simulink model "snap_sys_clk_feng"  (R2019a)
settings: Solver=VariableStepDiscrete  StartTime=0.0  StopTime=10.0  RelTol=1e-3
undefined symbols (not defined in the file): datetime, posixtime
libraries: xbsIndex_r4 x5252, casper_library_misc x69, xps_library x6, casper_library_delays x3
(part 39 of 45)

== system snap_sys_clk_feng/eq/pol1/conv_4bit/round4 ==
  din : Inport
  scale : Inport  Port=2
  Concat1 : xbsIndex_r4/Concat  num_inputs=2  dbl_ovrd=off  block_type=concat
      settings: block_version=10.1.3
  Concat2 : xbsIndex_r4/Concat  num_inputs=2  dbl_ovrd=off  block_type=concat
      settings: block_version=10.1.3
  Constant{,2,4,6} (4 alike) : xbsIndex_r4/Constant  const=(2^n_bits_out - 1) / 2^(n_bits_out)  gui_display_data_type=Fixed-point  arith_type=Signed (2's comp)  n_bits=n_bits_out  bin_pt=n_bits_out-1  preci_type=Single  exp_width=8  frac_width=24  explicit_period=on  period=1  equ=P=C  opselect=C  inp2=PCIN>>17  opr=+  inp1=P  carry=CIN  dbl_ovrd=off  block_type=constant
  Constant{1,3,5,7} (4 alike) : xbsIndex_r4/Constant  const=-(2^n_bits_out - 2) / 2^(n_bits_out)  gui_display_data_type=Fixed-point  arith_type=Signed (2's comp)  n_bits=n_bits_out  bin_pt=n_bits_out-1  preci_type=Single  exp_width=8  frac_width=24  explicit_period=on  period=1  equ=P=C  opselect=C  inp2=PCIN>>17  opr=+  inp1=P  carry=CIN  dbl_ovrd=off  block_type=constant
  Convert : xbsIndex_r4/Convert  gui_display_data_type=Fixed-point  arith_type="Signed  (2's comp)"  n_bits=n_bits_out  bin_pt=n_bits_out-1  float_type=Single  exp_bits=8  fraction_bits=24  quantization="Round  (unbiased: Even Values)"  overflow=Saturate  en=off  latency=5  pipeline=on  dbl_ovrd=off  block_type=convert
  Convert1 : xbsIndex_r4/Convert  gui_display_data_type=Fixed-point  arith_type="Signed  (2's comp)"  n_bits=n_bits_out  bin_pt=n_bits_out-1  float_type=Single  exp_bits=8  fraction_bits=24  quantization="Round  (unbiased: Even Values)"  overflow=Saturate  en=off  latency=5  pipeline=on  dbl_ovrd=off  block_type=convert
  Logical1 : xbsIndex_r4/Logical  logical_function=OR  inputs=4  en=off  latency=1  precision=Full  arith_type=Unsigned  n_bits=8  bin_pt=2  align_bp=on  dbl_ovrd=off  block_type=logical
      settings: xl_area=[0, 0, 0, 0, 0, 0, 0]
  Mult : xbsIndex_r4/Mult  precision=Full  arith_type="Signed  (2's comp)"  n_bits=8  bin_pt=2  quantization=Truncate  overflow=Wrap  en=off  latency=6  use_behavioral_HDL=off  opt=Speed  use_embedded=on  optimum_pipeline=off  pipeline=on  dbl_ovrd=off  use_rpm=on  placement_style=Rectangular shape  block_type=mult
      settings: xl_area=[0, 0, 0, 0, 0, 0, 0]  block_version=10.1.3
  Mult1 : xbsIndex_r4/Mult  precision=Full  arith_type="Signed  (2's comp)"  n_bits=8  bin_pt=2  quantization=Truncate  overflow=Wrap  en=off  latency=6  use_behavioral_HDL=off  opt=Speed  use_embedded=on  optimum_pipeline=on  pipeline=on  dbl_ovrd=off  use_rpm=on  placement_style=Rectangular shape  block_type=mult
      settings: xl_area=[0, 0, 0, 0, 0, 0, 0]  block_version=10.1.3
  Mux : xbsIndex_r4/Mux  inputs=3  en=off  latency=1  precision=Full  arith_type="Signed  (2's comp)"  n_bits=8  bin_pt=2  quantization=Truncate  overflow=Wrap  dbl_ovrd=off  block_type=mux
      settings: xl_area=[0, 0, 0, 0, 0, 0, 0]
  Mux1 : xbsIndex_r4/Mux  inputs=3  en=off  latency=1  precision=Full  arith_type="Signed  (2's comp)"  n_bits=8  bin_pt=2  quantization=Truncate  overflow=Wrap  dbl_ovrd=off  block_type=mux
      settings: xl_area=[0, 0, 0, 0, 0, 0, 0]
  Reinterpret4 : xbsIndex_r4/Reinterpret  force_arith_type=off  arith_type="Signed  (2's comp)"  force_bin_pt=on  bin_pt=coeff_bp  block_type=reinterpret
      settings: block_version=10.1.3
  Relational : xbsIndex_r4/Relational  mode=a>b  op_type=Bool  en=off  latency=5  dbl_ovrd=off  block_type=relational
      settings: xl_area=[0, 0, 0, 0, 0, 0, 0]  block_version=10.1.3
  Relational1 : xbsIndex_r4/Relational  mode=a<b  op_type=Bool  en=off  latency=5  dbl_ovrd=off  block_type=relational
      settings: xl_area=[0, 0, 0, 0, 0, 0, 0]  block_version=10.1.3
  Relational2 : xbsIndex_r4/Relational  mode=a>b  op_type=Bool  en=off  latency=5  dbl_ovrd=off  block_type=relational
      settings: xl_area=[0, 0, 0, 0, 0, 0, 0]  block_version=10.1.3
  Relational3 : xbsIndex_r4/Relational  mode=a<b  op_type=Bool  en=off  latency=5  dbl_ovrd=off  block_type=relational
      settings: xl_area=[0, 0, 0, 0, 0, 0, 0]  block_version=10.1.3
  c_to_ri : casper_library_misc/c_to_ri  n_bits=n_bits_in  bin_pt=n_bits_in-1
      settings: AttributesFormatString=25_24 r/i  SourceProductName=CASPER DSP Blockset
  ri_to_c : casper_library_misc/ri_to_c
      settings: SourceProductName=CASPER DSP Blockset
  dout : Outport
  clip : Outport  Port=2
  wires:
  din/1 -> c_to_ri/1
  ri_to_c/1 -> dout/1
  c_to_ri/1 -> Mult/1
  scale/1 -> Reinterpret4/1
  Convert/1 -> Mux/2
  Concat1/1 -> Mux/1
  Constant/1 -> Relational/2
  Constant1/1 -> Relational1/2
  Constant2/1 -> Mux/3
  Constant3/1 -> Mux/4
  Relational/1 -> Concat1/2, Logical1/1
  Relational1/1 -> Concat1/1, Logical1/2
  Concat2/1 -> Mux1/1
  Constant6/1 -> Mux1/3
  Constant7/1 -> Mux1/4
  Mux/1 -> ri_to_c/1
  Mux1/1 -> ri_to_c/2
  Mult/1 -> Convert/1, Relational/1, Relational1/1
  Logical1/1 -> clip/1
  Reinterpret4/1 -> Mult1/2, Mult/2
  Mult1/1 -> Relational3/1, Relational2/1, Convert1/1
  Constant5/1 -> Relational3/2
  Constant4/1 -> Relational2/2
  Convert1/1 -> Mux1/2
  Relational2/1 -> Logical1/3, Concat2/2
  Relational3/1 -> Logical1/4, Concat2/1
  c_to_ri/2 -> Mult1/1

== system snap_sys_clk_feng/eq/pol1/conv_8bit/bus_expand4 ==
  bus_in : Inport
  reinterpret{1..4} (4 alike) : xbsIndex_r4/Reinterpret  force_arith_type=on  arith_type=Unsigned  force_bin_pt=on  bin_pt=0  block_type=reinterpret
  slice1 : xbsIndex_r4/Slice  nbits=50  boolean_output=off  mode=Upper Bit Location + Width  bit1=-150  base1=MSB of Input  bit0=0  base0=LSB of Input  dbl_ovrd=off  block_type=slice
  slice2 : xbsIndex_r4/Slice  nbits=50  boolean_output=off  mode=Upper Bit Location + Width  bit1=-100  base1=MSB of Input  bit0=0  base0=LSB of Input  dbl_ovrd=off  block_type=slice
  slice3 : xbsIndex_r4/Slice  nbits=50  boolean_output=off  mode=Upper Bit Location + Width  bit1=-50  base1=MSB of Input  bit0=0  base0=LSB of Input  dbl_ovrd=off  block_type=slice
  slice4 : xbsIndex_r4/Slice  nbits=50  boolean_output=off  mode=Upper Bit Location + Width  bit1=0  base1=MSB of Input  bit0=0  base0=LSB of Input  dbl_ovrd=off  block_type=slice
  msb_out4 : Outport
  out3 : Outport  Port=2
  out2 : Outport  Port=3
  lsb_out1 : Outport  Port=4
  wires:
  bus_in/1 -> slice4/1, slice3/1, slice2/1, slice1/1
  slice4/1 -> reinterpret4/1
  reinterpret4/1 -> msb_out4/1
  slice3/1 -> reinterpret3/1
  reinterpret3/1 -> out3/1
  slice2/1 -> reinterpret2/1
  reinterpret2/1 -> out2/1
  slice1/1 -> reinterpret1/1
  reinterpret1/1 -> lsb_out1/1

== system snap_sys_clk_feng/eq/pol1/conv_8bit/round1 ==
  din : Inport
  scale : Inport  Port=2
  Concat1 : xbsIndex_r4/Concat  num_inputs=2  dbl_ovrd=off  block_type=concat
      settings: block_version=10.1.3
  Concat2 : xbsIndex_r4/Concat  num_inputs=2  dbl_ovrd=off  block_type=concat
      settings: block_version=10.1.3
  Constant{,2,4,6} (4 alike) : xbsIndex_r4/Constant  const=(2^n_bits_out - 1) / 2^(n_bits_out)  gui_display_data_type=Fixed-point  arith_type=Signed (2's comp)  n_bits=n_bits_out  bin_pt=n_bits_out-1  preci_type=Single  exp_width=8  frac_width=24  explicit_period=on  period=1  equ=P=C  opselect=C  inp2=PCIN>>17  opr=+  inp1=P  carry=CIN  dbl_ovrd=off  block_type=constant
  Constant{1,3,5,7} (4 alike) : xbsIndex_r4/Constant  const=-(2^n_bits_out - 2) / 2^(n_bits_out)  gui_display_data_type=Fixed-point  arith_type=Signed (2's comp)  n_bits=n_bits_out  bin_pt=n_bits_out-1  preci_type=Single  exp_width=8  frac_width=24  explicit_period=on  period=1  equ=P=C  opselect=C  inp2=PCIN>>17  opr=+  inp1=P  carry=CIN  dbl_ovrd=off  block_type=constant
  Convert : xbsIndex_r4/Convert  gui_display_data_type=Fixed-point  arith_type="Signed  (2's comp)"  n_bits=n_bits_out  bin_pt=n_bits_out-1  float_type=Single  exp_bits=8  fraction_bits=24  quantization="Round  (unbiased: Even Values)"  overflow=Saturate  en=off  latency=5  pipeline=on  dbl_ovrd=off  block_type=convert
  Convert1 : xbsIndex_r4/Convert  gui_display_data_type=Fixed-point  arith_type="Signed  (2's comp)"  n_bits=n_bits_out  bin_pt=n_bits_out-1  float_type=Single  exp_bits=8  fraction_bits=24  quantization="Round  (unbiased: Even Values)"  overflow=Saturate  en=off  latency=5  pipeline=on  dbl_ovrd=off  block_type=convert
  Logical1 : xbsIndex_r4/Logical  logical_function=OR  inputs=4  en=off  latency=1  precision=Full  arith_type=Unsigned  n_bits=8  bin_pt=2  align_bp=on  dbl_ovrd=off  block_type=logical
      settings: xl_area=[0, 0, 0, 0, 0, 0, 0]
  Mult : xbsIndex_r4/Mult  precision=Full  arith_type="Signed  (2's comp)"  n_bits=8  bin_pt=2  quantization=Truncate  overflow=Wrap  en=off  latency=6  use_behavioral_HDL=off  opt=Speed  use_embedded=on  optimum_pipeline=off  pipeline=on  dbl_ovrd=off  use_rpm=on  placement_style=Rectangular shape  block_type=mult
      settings: xl_area=[0, 0, 0, 0, 0, 0, 0]  block_version=10.1.3
  Mult1 : xbsIndex_r4/Mult  precision=Full  arith_type="Signed  (2's comp)"  n_bits=8  bin_pt=2  quantization=Truncate  overflow=Wrap  en=off  latency=6  use_behavioral_HDL=off  opt=Speed  use_embedded=on  optimum_pipeline=on  pipeline=on  dbl_ovrd=off  use_rpm=on  placement_style=Rectangular shape  block_type=mult
      settings: xl_area=[0, 0, 0, 0, 0, 0, 0]  block_version=10.1.3
  Mux : xbsIndex_r4/Mux  inputs=3  en=off  latency=1  precision=Full  arith_type="Signed  (2's comp)"  n_bits=8  bin_pt=2  quantization=Truncate  overflow=Wrap  dbl_ovrd=off  block_type=mux
      settings: xl_area=[0, 0, 0, 0, 0, 0, 0]
  Mux1 : xbsIndex_r4/Mux  inputs=3  en=off  latency=1  precision=Full  arith_type="Signed  (2's comp)"  n_bits=8  bin_pt=2  quantization=Truncate  overflow=Wrap  dbl_ovrd=off  block_type=mux
      settings: xl_area=[0, 0, 0, 0, 0, 0, 0]
  Reinterpret4 : xbsIndex_r4/Reinterpret  force_arith_type=off  arith_type="Signed  (2's comp)"  force_bin_pt=on  bin_pt=coeff_bp  block_type=reinterpret
      settings: block_version=10.1.3
  Relational : xbsIndex_r4/Relational  mode=a>b  op_type=Bool  en=off  latency=5  dbl_ovrd=off  block_type=relational
      settings: xl_area=[0, 0, 0, 0, 0, 0, 0]  block_version=10.1.3
  Relational1 : xbsIndex_r4/Relational  mode=a<b  op_type=Bool  en=off  latency=5  dbl_ovrd=off  block_type=relational
      settings: xl_area=[0, 0, 0, 0, 0, 0, 0]  block_version=10.1.3
  Relational2 : xbsIndex_r4/Relational  mode=a>b  op_type=Bool  en=off  latency=5  dbl_ovrd=off  block_type=relational
      settings: xl_area=[0, 0, 0, 0, 0, 0, 0]  block_version=10.1.3
  Relational3 : xbsIndex_r4/Relational  mode=a<b  op_type=Bool  en=off  latency=5  dbl_ovrd=off  block_type=relational
      settings: xl_area=[0, 0, 0, 0, 0, 0, 0]  block_version=10.1.3
  c_to_ri : casper_library_misc/c_to_ri  n_bits=n_bits_in  bin_pt=n_bits_in-1
      settings: AttributesFormatString=25_24 r/i  SourceProductName=CASPER DSP Blockset
  ri_to_c : casper_library_misc/ri_to_c
      settings: SourceProductName=CASPER DSP Blockset
  dout : Outport
  clip : Outport  Port=2
  wires:
  din/1 -> c_to_ri/1
  ri_to_c/1 -> dout/1
  c_to_ri/1 -> Mult/1
  scale/1 -> Reinterpret4/1
  Convert/1 -> Mux/2
  Concat1/1 -> Mux/1
  Constant/1 -> Relational/2
  Constant1/1 -> Relational1/2
  Constant2/1 -> Mux/3
  Constant3/1 -> Mux/4
  Relational/1 -> Concat1/2, Logical1/1
  Relational1/1 -> Concat1/1, Logical1/2
  Concat2/1 -> Mux1/1
  Constant6/1 -> Mux1/3
  Constant7/1 -> Mux1/4
  Mux/1 -> ri_to_c/1
  Mux1/1 -> ri_to_c/2
  Mult/1 -> Convert/1, Relational/1, Relational1/1
  Logical1/1 -> clip/1
  Reinterpret4/1 -> Mult1/2, Mult/2
  Mult1/1 -> Relational3/1, Relational2/1, Convert1/1
  Constant5/1 -> Relational3/2
  Constant4/1 -> Relational2/2
  Convert1/1 -> Mux1/2
  Relational2/1 -> Logical1/3, Concat2/2
  Relational3/1 -> Logical1/4, Concat2/1
  c_to_ri/2 -> Mult1/1

== system snap_sys_clk_feng/eq/pol1/conv_8bit/round2 ==
  din : Inport
  scale : Inport  Port=2
  Concat1 : xbsIndex_r4/Concat  num_inputs=2  dbl_ovrd=off  block_type=concat
      settings: block_version=10.1.3
  Concat2 : xbsIndex_r4/Concat  num_inputs=2  dbl_ovrd=off  block_type=concat
      settings: block_version=10.1.3
  Constant{,2,4,6} (4 alike) : xbsIndex_r4/Constant  const=(2^n_bits_out - 1) / 2^(n_bits_out)  gui_display_data_type=Fixed-point  arith_type=Signed (2's comp)  n_bits=n_bits_out  bin_pt=n_bits_out-1  preci_type=Single  exp_width=8  frac_width=24  explicit_period=on  period=1  equ=P=C  opselect=C  inp2=PCIN>>17  opr=+  inp1=P  carry=CIN  dbl_ovrd=off  block_type=constant
  Constant{1,3,5,7} (4 alike) : xbsIndex_r4/Constant  const=-(2^n_bits_out - 2) / 2^(n_bits_out)  gui_display_data_type=Fixed-point  arith_type=Signed (2's comp)  n_bits=n_bits_out  bin_pt=n_bits_out-1  preci_type=Single  exp_width=8  frac_width=24  explicit_period=on  period=1  equ=P=C  opselect=C  inp2=PCIN>>17  opr=+  inp1=P  carry=CIN  dbl_ovrd=off  block_type=constant
  Convert : xbsIndex_r4/Convert  gui_display_data_type=Fixed-point  arith_type="Signed  (2's comp)"  n_bits=n_bits_out  bin_pt=n_bits_out-1  float_type=Single  exp_bits=8  fraction_bits=24  quantization="Round  (unbiased: Even Values)"  overflow=Saturate  en=off  latency=5  pipeline=on  dbl_ovrd=off  block_type=convert
  Convert1 : xbsIndex_r4/Convert  gui_display_data_type=Fixed-point  arith_type="Signed  (2's comp)"  n_bits=n_bits_out  bin_pt=n_bits_out-1  float_type=Single  exp_bits=8  fraction_bits=24  quantization="Round  (unbiased: Even Values)"  overflow=Saturate  en=off  latency=5  pipeline=on  dbl_ovrd=off  block_type=convert
  Logical1 : xbsIndex_r4/Logical  logical_function=OR  inputs=4  en=off  latency=1  precision=Full  arith_type=Unsigned  n_bits=8  bin_pt=2  align_bp=on  dbl_ovrd=off  block_type=logical
      settings: xl_area=[0, 0, 0, 0, 0, 0, 0]
  Mult : xbsIndex_r4/Mult  precision=Full  arith_type="Signed  (2's comp)"  n_bits=8  bin_pt=2  quantization=Truncate  overflow=Wrap  en=off  latency=6  use_behavioral_HDL=off  opt=Speed  use_embedded=on  optimum_pipeline=off  pipeline=on  dbl_ovrd=off  use_rpm=on  placement_style=Rectangular shape  block_type=mult
      settings: xl_area=[0, 0, 0, 0, 0, 0, 0]  block_version=10.1.3
  Mult1 : xbsIndex_r4/Mult  precision=Full  arith_type="Signed  (2's comp)"  n_bits=8  bin_pt=2  quantization=Truncate  overflow=Wrap  en=off  latency=6  use_behavioral_HDL=off  opt=Speed  use_embedded=on  optimum_pipeline=on  pipeline=on  dbl_ovrd=off  use_rpm=on  placement_style=Rectangular shape  block_type=mult
      settings: xl_area=[0, 0, 0, 0, 0, 0, 0]  block_version=10.1.3
  Mux : xbsIndex_r4/Mux  inputs=3  en=off  latency=1  precision=Full  arith_type="Signed  (2's comp)"  n_bits=8  bin_pt=2  quantization=Truncate  overflow=Wrap  dbl_ovrd=off  block_type=mux
      settings: xl_area=[0, 0, 0, 0, 0, 0, 0]
  Mux1 : xbsIndex_r4/Mux  inputs=3  en=off  latency=1  precision=Full  arith_type="Signed  (2's comp)"  n_bits=8  bin_pt=2  quantization=Truncate  overflow=Wrap  dbl_ovrd=off  block_type=mux
      settings: xl_area=[0, 0, 0, 0, 0, 0, 0]
  Reinterpret4 : xbsIndex_r4/Reinterpret  force_arith_type=off  arith_type="Signed  (2's comp)"  force_bin_pt=on  bin_pt=coeff_bp  block_type=reinterpret
      settings: block_version=10.1.3
  Relational : xbsIndex_r4/Relational  mode=a>b  op_type=Bool  en=off  latency=5  dbl_ovrd=off  block_type=relational
      settings: xl_area=[0, 0, 0, 0, 0, 0, 0]  block_version=10.1.3
  Relational1 : xbsIndex_r4/Relational  mode=a<b  op_type=Bool  en=off  latency=5  dbl_ovrd=off  block_type=relational
      settings: xl_area=[0, 0, 0, 0, 0, 0, 0]  block_version=10.1.3
  Relational2 : xbsIndex_r4/Relational  mode=a>b  op_type=Bool  en=off  latency=5  dbl_ovrd=off  block_type=relational
      settings: xl_area=[0, 0, 0, 0, 0, 0, 0]  block_version=10.1.3
  Relational3 : xbsIndex_r4/Relational  mode=a<b  op_type=Bool  en=off  latency=5  dbl_ovrd=off  block_type=relational
      settings: xl_area=[0, 0, 0, 0, 0, 0, 0]  block_version=10.1.3
  c_to_ri : casper_library_misc/c_to_ri  n_bits=n_bits_in  bin_pt=n_bits_in-1
      settings: AttributesFormatString=25_24 r/i  SourceProductName=CASPER DSP Blockset
  ri_to_c : casper_library_misc/ri_to_c
      settings: SourceProductName=CASPER DSP Blockset
  dout : Outport
  clip : Outport  Port=2
  wires:
  c_to_ri/2 -> Mult1/1
  Relational3/1 -> Concat2/1, Logical1/4
  Relational2/1 -> Concat2/2, Logical1/3
  Convert1/1 -> Mux1/2
  Constant4/1 -> Relational2/2
  Constant5/1 -> Relational3/2
  Mult1/1 -> Convert1/1, Relational2/1, Relational3/1
  Reinterpret4/1 -> Mult/2, Mult1/2
  Logical1/1 -> clip/1
  Mult/1 -> Relational1/1, Relational/1, Convert/1
  Mux1/1 -> ri_to_c/2
  Mux/1 -> ri_to_c/1
  Constant7/1 -> Mux1/4
  Constant6/1 -> Mux1/3
  Concat2/1 -> Mux1/1
  Relational1/1 -> Logical1/2, Concat1/1
  Relational/1 -> Logical1/1, Concat1/2
  Constant3/1 -> Mux/4
  Constant2/1 -> Mux/3
  Constant1/1 -> Relational1/2
  Constant/1 -> Relational/2
  Concat1/1 -> Mux/1
  Convert/1 -> Mux/2
  scale/1 -> Reinterpret4/1
  c_to_ri/1 -> Mult/1
  ri_to_c/1 -> dout/1
  din/1 -> c_to_ri/1

== system snap_sys_clk_feng/eq/pol1/conv_8bit/round3 ==
  din : Inport
  scale : Inport  Port=2
  Concat1 : xbsIndex_r4/Concat  num_inputs=2  dbl_ovrd=off  block_type=concat
      settings: block_version=10.1.3
  Concat2 : xbsIndex_r4/Concat  num_inputs=2  dbl_ovrd=off  block_type=concat
      settings: block_version=10.1.3
  Constant{,2,4,6} (4 alike) : xbsIndex_r4/Constant  const=(2^n_bits_out - 1) / 2^(n_bits_out)  gui_display_data_type=Fixed-point  arith_type=Signed (2's comp)  n_bits=n_bits_out  bin_pt=n_bits_out-1  preci_type=Single  exp_width=8  frac_width=24  explicit_period=on  period=1  equ=P=C  opselect=C  inp2=PCIN>>17  opr=+  inp1=P  carry=CIN  dbl_ovrd=off  block_type=constant
  Constant{1,3,5,7} (4 alike) : xbsIndex_r4/Constant  const=-(2^n_bits_out - 2) / 2^(n_bits_out)  gui_display_data_type=Fixed-point  arith_type=Signed (2's comp)  n_bits=n_bits_out  bin_pt=n_bits_out-1  preci_type=Single  exp_width=8  frac_width=24  explicit_period=on  period=1  equ=P=C  opselect=C  inp2=PCIN>>17  opr=+  inp1=P  carry=CIN  dbl_ovrd=off  block_type=constant
  Convert : xbsIndex_r4/Convert  gui_display_data_type=Fixed-point  arith_type="Signed  (2's comp)"  n_bits=n_bits_out  bin_pt=n_bits_out-1  float_type=Single  exp_bits=8  fraction_bits=24  quantization="Round  (unbiased: Even Values)"  overflow=Saturate  en=off  latency=5  pipeline=on  dbl_ovrd=off  block_type=convert
  Convert1 : xbsIndex_r4/Convert  gui_display_data_type=Fixed-point  arith_type="Signed  (2's comp)"  n_bits=n_bits_out  bin_pt=n_bits_out-1  float_type=Single  exp_bits=8  fraction_bits=24  quantization="Round  (unbiased: Even Values)"  overflow=Saturate  en=off  latency=5  pipeline=on  dbl_ovrd=off  block_type=convert
  Logical1 : xbsIndex_r4/Logical  logical_function=OR  inputs=4  en=off  latency=1  precision=Full  arith_type=Unsigned  n_bits=8  bin_pt=2  align_bp=on  dbl_ovrd=off  block_type=logical
      settings: xl_area=[0, 0, 0, 0, 0, 0, 0]
  Mult : xbsIndex_r4/Mult  precision=Full  arith_type="Signed  (2's comp)"  n_bits=8  bin_pt=2  quantization=Truncate  overflow=Wrap  en=off  latency=6  use_behavioral_HDL=off  opt=Speed  use_embedded=on  optimum_pipeline=off  pipeline=on  dbl_ovrd=off  use_rpm=on  placement_style=Rectangular shape  block_type=mult
      settings: xl_area=[0, 0, 0, 0, 0, 0, 0]  block_version=10.1.3
  Mult1 : xbsIndex_r4/Mult  precision=Full  arith_type="Signed  (2's comp)"  n_bits=8  bin_pt=2  quantization=Truncate  overflow=Wrap  en=off  latency=6  use_behavioral_HDL=off  opt=Speed  use_embedded=on  optimum_pipeline=on  pipeline=on  dbl_ovrd=off  use_rpm=on  placement_style=Rectangular shape  block_type=mult
      settings: xl_area=[0, 0, 0, 0, 0, 0, 0]  block_version=10.1.3
  Mux : xbsIndex_r4/Mux  inputs=3  en=off  latency=1  precision=Full  arith_type="Signed  (2's comp)"  n_bits=8  bin_pt=2  quantization=Truncate  overflow=Wrap  dbl_ovrd=off  block_type=mux
      settings: xl_area=[0, 0, 0, 0, 0, 0, 0]
  Mux1 : xbsIndex_r4/Mux  inputs=3  en=off  latency=1  precision=Full  arith_type="Signed  (2's comp)"  n_bits=8  bin_pt=2  quantization=Truncate  overflow=Wrap  dbl_ovrd=off  block_type=mux
      settings: xl_area=[0, 0, 0, 0, 0, 0, 0]
  Reinterpret4 : xbsIndex_r4/Reinterpret  force_arith_type=off  arith_type="Signed  (2's comp)"  force_bin_pt=on  bin_pt=coeff_bp  block_type=reinterpret
      settings: block_version=10.1.3
  Relational : xbsIndex_r4/Relational  mode=a>b  op_type=Bool  en=off  latency=5  dbl_ovrd=off  block_type=relational
      settings: xl_area=[0, 0, 0, 0, 0, 0, 0]  block_version=10.1.3
  Relational1 : xbsIndex_r4/Relational  mode=a<b  op_type=Bool  en=off  latency=5  dbl_ovrd=off  block_type=relational
      settings: xl_area=[0, 0, 0, 0, 0, 0, 0]  block_version=10.1.3
  Relational2 : xbsIndex_r4/Relational  mode=a>b  op_type=Bool  en=off  latency=5  dbl_ovrd=off  block_type=relational
      settings: xl_area=[0, 0, 0, 0, 0, 0, 0]  block_version=10.1.3
  Relational3 : xbsIndex_r4/Relational  mode=a<b  op_type=Bool  en=off  latency=5  dbl_ovrd=off  block_type=relational
      settings: xl_area=[0, 0, 0, 0, 0, 0, 0]  block_version=10.1.3
  c_to_ri : casper_library_misc/c_to_ri  n_bits=n_bits_in  bin_pt=n_bits_in-1
      settings: AttributesFormatString=25_24 r/i  SourceProductName=CASPER DSP Blockset
  ri_to_c : casper_library_misc/ri_to_c
      settings: SourceProductName=CASPER DSP Blockset
  dout : Outport
  clip : Outport  Port=2
  wires:
  din/1 -> c_to_ri/1
  ri_to_c/1 -> dout/1
  c_to_ri/1 -> Mult/1
  scale/1 -> Reinterpret4/1
  Convert/1 -> Mux/2
  Concat1/1 -> Mux/1
  Constant/1 -> Relational/2
  Constant1/1 -> Relational1/2
  Constant2/1 -> Mux/3
  Constant3/1 -> Mux/4
  Relational/1 -> Concat1/2, Logical1/1
  Relational1/1 -> Concat1/1, Logical1/2
  Concat2/1 -> Mux1/1
  Constant6/1 -> Mux1/3
  Constant7/1 -> Mux1/4
  Mux/1 -> ri_to_c/1
  Mux1/1 -> ri_to_c/2
  Mult/1 -> Convert/1, Relational/1, Relational1/1
  Logical1/1 -> clip/1
  Reinterpret4/1 -> Mult1/2, Mult/2
  Mult1/1 -> Relational3/1, Relational2/1, Convert1/1
  Constant5/1 -> Relational3/2
  Constant4/1 -> Relational2/2
  Convert1/1 -> Mux1/2
  Relational2/1 -> Logical1/3, Concat2/2
  Relational3/1 -> Logical1/4, Concat2/1
  c_to_ri/2 -> Mult1/1

== system snap_sys_clk_feng/eq/pol1/conv_8bit/round4 ==
  din : Inport
  scale : Inport  Port=2
  Concat1 : xbsIndex_r4/Concat  num_inputs=2  dbl_ovrd=off  block_type=concat
      settings: block_version=10.1.3
  Concat2 : xbsIndex_r4/Concat  num_inputs=2  dbl_ovrd=off  block_type=concat
      settings: block_version=10.1.3
  Constant{,2,4,6} (4 alike) : xbsIndex_r4/Constant  const=(2^n_bits_out - 1) / 2^(n_bits_out)  gui_display_data_type=Fixed-point  arith_type=Signed (2's comp)  n_bits=n_bits_out  bin_pt=n_bits_out-1  preci_type=Single  exp_width=8  frac_width=24  explicit_period=on  period=1  equ=P=C  opselect=C  inp2=PCIN>>17  opr=+  inp1=P  carry=CIN  dbl_ovrd=off  block_type=constant
  Constant{1,3,5,7} (4 alike) : xbsIndex_r4/Constant  const=-(2^n_bits_out - 2) / 2^(n_bits_out)  gui_display_data_type=Fixed-point  arith_type=Signed (2's comp)  n_bits=n_bits_out  bin_pt=n_bits_out-1  preci_type=Single  exp_width=8  frac_width=24  explicit_period=on  period=1  equ=P=C  opselect=C  inp2=PCIN>>17  opr=+  inp1=P  carry=CIN  dbl_ovrd=off  block_type=constant
  Convert : xbsIndex_r4/Convert  gui_display_data_type=Fixed-point  arith_type="Signed  (2's comp)"  n_bits=n_bits_out  bin_pt=n_bits_out-1  float_type=Single  exp_bits=8  fraction_bits=24  quantization="Round  (unbiased: Even Values)"  overflow=Saturate  en=off  latency=5  pipeline=on  dbl_ovrd=off  block_type=convert
  Convert1 : xbsIndex_r4/Convert  gui_display_data_type=Fixed-point  arith_type="Signed  (2's comp)"  n_bits=n_bits_out  bin_pt=n_bits_out-1  float_type=Single  exp_bits=8  fraction_bits=24  quantization="Round  (unbiased: Even Values)"  overflow=Saturate  en=off  latency=5  pipeline=on  dbl_ovrd=off  block_type=convert
  Logical1 : xbsIndex_r4/Logical  logical_function=OR  inputs=4  en=off  latency=1  precision=Full  arith_type=Unsigned  n_bits=8  bin_pt=2  align_bp=on  dbl_ovrd=off  block_type=logical
      settings: xl_area=[0, 0, 0, 0, 0, 0, 0]
  Mult : xbsIndex_r4/Mult  precision=Full  arith_type="Signed  (2's comp)"  n_bits=8  bin_pt=2  quantization=Truncate  overflow=Wrap  en=off  latency=6  use_behavioral_HDL=off  opt=Speed  use_embedded=on  optimum_pipeline=off  pipeline=on  dbl_ovrd=off  use_rpm=on  placement_style=Rectangular shape  block_type=mult
      settings: xl_area=[0, 0, 0, 0, 0, 0, 0]  block_version=10.1.3
  Mult1 : xbsIndex_r4/Mult  precision=Full  arith_type="Signed  (2's comp)"  n_bits=8  bin_pt=2  quantization=Truncate  overflow=Wrap  en=off  latency=6  use_behavioral_HDL=off  opt=Speed  use_embedded=on  optimum_pipeline=on  pipeline=on  dbl_ovrd=off  use_rpm=on  placement_style=Rectangular shape  block_type=mult
      settings: xl_area=[0, 0, 0, 0, 0, 0, 0]  block_version=10.1.3
  Mux : xbsIndex_r4/Mux  inputs=3  en=off  latency=1  precision=Full  arith_type="Signed  (2's comp)"  n_bits=8  bin_pt=2  quantization=Truncate  overflow=Wrap  dbl_ovrd=off  block_type=mux
      settings: xl_area=[0, 0, 0, 0, 0, 0, 0]
  Mux1 : xbsIndex_r4/Mux  inputs=3  en=off  latency=1  precision=Full  arith_type="Signed  (2's comp)"  n_bits=8  bin_pt=2  quantization=Truncate  overflow=Wrap  dbl_ovrd=off  block_type=mux
      settings: xl_area=[0, 0, 0, 0, 0, 0, 0]
  Reinterpret4 : xbsIndex_r4/Reinterpret  force_arith_type=off  arith_type="Signed  (2's comp)"  force_bin_pt=on  bin_pt=coeff_bp  block_type=reinterpret
      settings: block_version=10.1.3
  Relational : xbsIndex_r4/Relational  mode=a>b  op_type=Bool  en=off  latency=5  dbl_ovrd=off  block_type=relational
      settings: xl_area=[0, 0, 0, 0, 0, 0, 0]  block_version=10.1.3
  Relational1 : xbsIndex_r4/Relational  mode=a<b  op_type=Bool  en=off  latency=5  dbl_ovrd=off  block_type=relational
      settings: xl_area=[0, 0, 0, 0, 0, 0, 0]  block_version=10.1.3
  Relational2 : xbsIndex_r4/Relational  mode=a>b  op_type=Bool  en=off  latency=5  dbl_ovrd=off  block_type=relational
      settings: xl_area=[0, 0, 0, 0, 0, 0, 0]  block_version=10.1.3
  Relational3 : xbsIndex_r4/Relational  mode=a<b  op_type=Bool  en=off  latency=5  dbl_ovrd=off  block_type=relational
      settings: xl_area=[0, 0, 0, 0, 0, 0, 0]  block_version=10.1.3
  c_to_ri : casper_library_misc/c_to_ri  n_bits=n_bits_in  bin_pt=n_bits_in-1
      settings: AttributesFormatString=25_24 r/i  SourceProductName=CASPER DSP Blockset
  ri_to_c : casper_library_misc/ri_to_c
      settings: SourceProductName=CASPER DSP Blockset
  dout : Outport
  clip : Outport  Port=2
  wires:
  c_to_ri/2 -> Mult1/1
  Relational3/1 -> Concat2/1, Logical1/4
  Relational2/1 -> Concat2/2, Logical1/3
  Convert1/1 -> Mux1/2
  Constant4/1 -> Relational2/2
  Constant5/1 -> Relational3/2
  Mult1/1 -> Convert1/1, Relational2/1, Relational3/1
  Reinterpret4/1 -> Mult/2, Mult1/2
  Logical1/1 -> clip/1
  Mult/1 -> Relational1/1, Relational/1, Convert/1
  Mux1/1 -> ri_to_c/2
  Mux/1 -> ri_to_c/1
  Constant7/1 -> Mux1/4
  Constant6/1 -> Mux1/3
  Concat2/1 -> Mux1/1
  Relational1/1 -> Logical1/2, Concat1/1
  Relational/1 -> Logical1/1, Concat1/2
  Constant3/1 -> Mux/4
  Constant2/1 -> Mux/3
  Constant1/1 -> Relational1/2
  Constant/1 -> Relational/2
  Concat1/1 -> Mux/1
  Convert/1 -> Mux/2
  scale/1 -> Reinterpret4/1
  c_to_ri/1 -> Mult/1
  ri_to_c/1 -> dout/1
  din/1 -> c_to_ri/1

== system snap_sys_clk_feng/eqtvg/pol0/tv/calc_add ==
  note: If reading/writing words
      | smaller than 32 bits,
      | change address so
      | that addressing is
      | big endian instead of
      | little, otherwise
      | pass through
  note: Use behavioural HDL
      | so that gets optimised
      | to minimum logic
  in : Inport
  add_sub : xbsIndex_r4/AddSub  mode=Subtraction  use_carryin=off  use_carryout=off  en=off  latency=0  precision=User Defined  arith_type=Unsigned  n_bits=max(1, log2(32/data_width))  bin_pt=0  quantization=Truncate  overflow=Wrap  use_behavioral_HDL=on  hw_selection=Fabric  pipelined=off  dbl_ovrd=off  block_type=addsub
  concat : xbsIndex_r4/Concat  num_inputs=2  dbl_ovrd=off  block_type=concat
  const : xbsIndex_r4/Constant  const=max(0, 32/data_width-1)  gui_display_data_type=Fixed-point  arith_type=Unsigned  n_bits=max(1, log2(32/data_width))  bin_pt=0  preci_type=Single  exp_width=8  frac_width=24  explicit_period=on  period=sample_rate  equ=P=C  opselect=C  inp2=PCIN>>17  opr=+  inp1=P  carry=CIN  dbl_ovrd=off  block_type=constant
      settings: block_version=11.4
  convert_addr : xbsIndex_r4/Convert  gui_display_data_type=Fixed-point  arith_type=Unsigned  n_bits=addr_width  bin_pt=0  float_type=Single  exp_bits=8  fraction_bits=24  quantization=Truncate  overflow=Wrap  en=off  latency=0  pipeline=off  dbl_ovrd=off  block_type=convert
      settings: xl_area=[0, 0, 0, 0, 0, 0, 0]
  lsw : xbsIndex_r4/Slice  nbits=max(1, log2(32/data_width))  boolean_output=off  mode=Lower Bit Location + Width  bit1=0  base1=MSB of Input  bit0=0  base0=LSB of Input  dbl_ovrd=off  block_type=slice
  manipulate : xbsIndex_r4/Constant  const=min(1, floor(32/data_width) - 1)  gui_display_data_type=Fixed-point  arith_type=Unsigned  n_bits=1  bin_pt=0  preci_type=Single  exp_width=8  frac_width=24  explicit_period=on  period=sample_rate  equ=P=C  opselect=C  inp2=PCIN>>17  opr=+  inp1=P  carry=CIN  dbl_ovrd=off  block_type=constant
      settings: block_version=11.4
  msw : xbsIndex_r4/Slice  nbits=addr_width - max(1, log2(32/data_width))  boolean_output=off  mode=Upper Bit Location + Width  bit1=0  base1=MSB of Input  bit0=0  base0=LSB of Input  dbl_ovrd=off  block_type=slice
  mux : xbsIndex_r4/Mux  inputs=2  en=off  latency=0  precision=Full  arith_type=Unsigned  n_bits=16  bin_pt=14  quantization=Truncate  overflow=Wrap  dbl_ovrd=off  block_type=mux
      settings: block_version=11.4
  out : Outport
  wires:
  in/1 -> convert_addr/1
  add_sub/1 -> concat/2
  msw/1 -> concat/1
  concat/1 -> mux/3
  manipulate/1 -> mux/1
  mux/1 -> out/1
  lsw/1 -> add_sub/2
  const/1 -> add_sub/1
  convert_addr/1 -> lsw/1, msw/1, mux/2

== system snap_sys_clk_feng/eqtvg/pol0/tv/munge_in ==
  din : Inport
  reinterpret_out : xbsIndex_r4/Reinterpret  force_arith_type=on  arith_type=Unsigned  force_bin_pt=on  bin_pt=0  block_type=reinterpret
  dout : Outport
  wires:
  reinterpret_out/1 -> dout/1
  din/1 -> reinterpret_out/1

== system snap_sys_clk_feng/eqtvg/pol0/tv/munge_out ==
  din : Inport
  reinterpret_out : xbsIndex_r4/Reinterpret  force_arith_type=on  arith_type=Unsigned  force_bin_pt=on  bin_pt=0  block_type=reinterpret
  dout : Outport
  wires:
  reinterpret_out/1 -> dout/1
  din/1 -> reinterpret_out/1

== system snap_sys_clk_feng/eqtvg/pol0/tv/sim_mem ==
  addr : Inport
  data : Inport  Port=2
  we : Inport  Port=3
  Data Type Conversion : DataTypeConversion  OutDataTypeStr=single
  Data Type Conversion1 : DataTypeConversion  OutDataTypeStr=double
  Data Type Conversion2 : DataTypeConversion  OutDataTypeStr=boolean
  sfunc : M-S-Function  FunctionName=shared_bram_sim_sfunc  Parameters=depth_bits, latency, init_vals  mask{depth_bits=addr_width, latency=csp_latency, init_vals=init_vals}
      mask prompts: depth_bits "Depth (2^?):"; latency "Latency (>=1):"; init_vals "Initial values:"
      mask Callback latency:
      | latency = str2double(get_param(gcb, 'latency'));
      | if latency < 1
      |     errordlg('Cannot have latency less than one.');
      |     set_param(gcb, 'latency', '1');
      | end
  sim_addr : xbsIndex_r4/Gateway Out  inherit_from_input=off  hdl_port=off  rows=1  columns=1  UseAsDAC=off  DACChannel='1'  interface=None  automatic_assignment=on  address_offset=hex2dec('00')  intf_name=''  intf_description=''  timing_constraint=None  locs_specified=off  LOCs={}  io_standard={}  block_type=gatewayout
  sim_data : xbsIndex_r4/Gateway Out  inherit_from_input=off  hdl_port=off  rows=1  columns=1  UseAsDAC=off  DACChannel='1'  interface=None  automatic_assignment=on  address_offset=hex2dec('00')  intf_name=''  intf_description=''  timing_constraint=None  locs_specified=off  LOCs={}  io_standard={}  block_type=gatewayout
  sim_we : xbsIndex_r4/Gateway Out  inherit_from_input=off  hdl_port=off  rows=1  columns=1  UseAsDAC=off  DACChannel='1'  interface=None  automatic_assignment=on  address_offset=hex2dec('00')  intf_name=''  intf_description=''  timing_constraint=None  locs_specified=off  LOCs={}  io_standard={}  block_type=gatewayout
  data_out : Outport
  wires:
  addr/1 -> sim_addr/1
  data/1 -> sim_data/1
  we/1 -> sim_we/1
  sim_addr/1 -> Data Type Conversion/1
  sim_data/1 -> Data Type Conversion1/1
  sim_we/1 -> Data Type Conversion2/1
  Data Type Conversion/1 -> sfunc/1  "addr"
  Data Type Conversion1/1 -> sfunc/2  "data_in"
  Data Type Conversion2/1 -> sfunc/3  "we"
  sfunc/1 -> data_out/1  "output"

== system snap_sys_clk_feng/eqtvg/pol1/tv/calc_add ==
  note: Use behavioural HDL
      | so that gets optimised
      | to minimum logic
  note: If reading/writing words
      | smaller than 32 bits,
      | change address so
      | that addressing is
      | big endian instead of
      | little, otherwise
      | pass through
  in : Inport
  add_sub : xbsIndex_r4/AddSub  mode=Subtraction  use_carryin=off  use_carryout=off  en=off  latency=0  precision=User Defined  arith_type=Unsigned  n_bits=max(1, log2(32/data_width))  bin_pt=0  quantization=Truncate  overflow=Wrap  use_behavioral_HDL=on  hw_selection=Fabric  pipelined=off  dbl_ovrd=off  block_type=addsub
  concat : xbsIndex_r4/Concat  num_inputs=2  dbl_ovrd=off  block_type=concat
  const : xbsIndex_r4/Constant  const=max(0, 32/data_width-1)  gui_display_data_type=Fixed-point  arith_type=Unsigned  n_bits=max(1, log2(32/data_width))  bin_pt=0  preci_type=Single  exp_width=8  frac_width=24  explicit_period=on  period=sample_rate  equ=P=C  opselect=C  inp2=PCIN>>17  opr=+  inp1=P  carry=CIN  dbl_ovrd=off  block_type=constant
      settings: block_version=11.4
  convert_addr : xbsIndex_r4/Convert  gui_display_data_type=Fixed-point  arith_type=Unsigned  n_bits=addr_width  bin_pt=0  float_type=Single  exp_bits=8  fraction_bits=24  quantization=Truncate  overflow=Wrap  en=off  latency=0  pipeline=off  dbl_ovrd=off  block_type=convert
      settings: xl_area=[0, 0, 0, 0, 0, 0, 0]
  lsw : xbsIndex_r4/Slice  nbits=max(1, log2(32/data_width))  boolean_output=off  mode=Lower Bit Location + Width  bit1=0  base1=MSB of Input  bit0=0  base0=LSB of Input  dbl_ovrd=off  block_type=slice
  manipulate : xbsIndex_r4/Constant  const=min(1, floor(32/data_width) - 1)  gui_display_data_type=Fixed-point  arith_type=Unsigned  n_bits=1  bin_pt=0  preci_type=Single  exp_width=8  frac_width=24  explicit_period=on  period=sample_rate  equ=P=C  opselect=C  inp2=PCIN>>17  opr=+  inp1=P  carry=CIN  dbl_ovrd=off  block_type=constant
      settings: block_version=11.4
  msw : xbsIndex_r4/Slice  nbits=addr_width - max(1, log2(32/data_width))  boolean_output=off  mode=Upper Bit Location + Width  bit1=0  base1=MSB of Input  bit0=0  base0=LSB of Input  dbl_ovrd=off  block_type=slice
  mux : xbsIndex_r4/Mux  inputs=2  en=off  latency=0  precision=Full  arith_type=Unsigned  n_bits=16  bin_pt=14  quantization=Truncate  overflow=Wrap  dbl_ovrd=off  block_type=mux
      settings: block_version=11.4
  out : Outport
  wires:
  convert_addr/1 -> mux/2, msw/1, lsw/1
  const/1 -> add_sub/1
  lsw/1 -> add_sub/2
  mux/1 -> out/1
  manipulate/1 -> mux/1
  concat/1 -> mux/3
  msw/1 -> concat/1
  add_sub/1 -> concat/2
  in/1 -> convert_addr/1

== system snap_sys_clk_feng/eqtvg/pol1/tv/munge_in ==
  din : Inport
  reinterpret_out : xbsIndex_r4/Reinterpret  force_arith_type=on  arith_type=Unsigned  force_bin_pt=on  bin_pt=0  block_type=reinterpret
  dout : Outport
  wires:
  din/1 -> reinterpret_out/1
  reinterpret_out/1 -> dout/1

== system snap_sys_clk_feng/eqtvg/pol1/tv/munge_out ==
  din : Inport
  reinterpret_out : xbsIndex_r4/Reinterpret  force_arith_type=on  arith_type=Unsigned  force_bin_pt=on  bin_pt=0  block_type=reinterpret
  dout : Outport
  wires:
  din/1 -> reinterpret_out/1
  reinterpret_out/1 -> dout/1

== system snap_sys_clk_feng/eqtvg/pol1/tv/sim_mem ==
  addr : Inport
  data : Inport  Port=2
  we : Inport  Port=3
  Data Type Conversion : DataTypeConversion  OutDataTypeStr=single
  Data Type Conversion1 : DataTypeConversion  OutDataTypeStr=double
  Data Type Conversion2 : DataTypeConversion  OutDataTypeStr=boolean
  sfunc : M-S-Function  FunctionName=shared_bram_sim_sfunc  Parameters=depth_bits, latency, init_vals  mask{depth_bits=addr_width, latency=csp_latency, init_vals=init_vals}
      mask prompts: depth_bits "Depth (2^?):"; latency "Latency (>=1):"; init_vals "Initial values:"
      mask Callback latency:
      | latency = str2double(get_param(gcb, 'latency'));
      | if latency < 1
      |     errordlg('Cannot have latency less than one.');
      |     set_param(gcb, 'latency', '1');
      | end
  sim_addr : xbsIndex_r4/Gateway Out  inherit_from_input=off  hdl_port=off  rows=1  columns=1  UseAsDAC=off  DACChannel='1'  interface=None  automatic_assignment=on  address_offset=hex2dec('00')  intf_name=''  intf_description=''  timing_constraint=None  locs_specified=off  LOCs={}  io_standard={}  block_type=gatewayout
  sim_data : xbsIndex_r4/Gateway Out  inherit_from_input=off  hdl_port=off  rows=1  columns=1  UseAsDAC=off  DACChannel='1'  interface=None  automatic_assignment=on  address_offset=hex2dec('00')  intf_name=''  intf_description=''  timing_constraint=None  locs_specified=off  LOCs={}  io_standard={}  block_type=gatewayout
  sim_we : xbsIndex_r4/Gateway Out  inherit_from_input=off  hdl_port=off  rows=1  columns=1  UseAsDAC=off  DACChannel='1'  interface=None  automatic_assignment=on  address_offset=hex2dec('00')  intf_name=''  intf_description=''  timing_constraint=None  locs_specified=off  LOCs={}  io_standard={}  block_type=gatewayout
  data_out : Outport
  wires:
  sfunc/1 -> data_out/1  "output"
  Data Type Conversion2/1 -> sfunc/3  "we"
  Data Type Conversion1/1 -> sfunc/2  "data_in"
  Data Type Conversion/1 -> sfunc/1  "addr"
  sim_we/1 -> Data Type Conversion2/1
  sim_data/1 -> Data Type Conversion1/1
  sim_addr/1 -> Data Type Conversion/1
  we/1 -> sim_we/1
  data/1 -> sim_data/1
  addr/1 -> sim_addr/1

== system snap_sys_clk_feng/packetizer0/header/munge_in/join ==
  in1 : Inport
  in2 : Inport  Port=2
  concatenate : xbsIndex_r4/Concat  num_inputs=2  dbl_ovrd=off  block_type=concat
  reinterpret1 : xbsIndex_r4/Reinterpret  force_arith_type=on  arith_type=Unsigned  force_bin_pt=on  bin_pt=0  block_type=reinterpret
      settings: infoedit="Changes signal type without altering the binary representation.   You can changed the signal between signed and unsigned, and relocate the binary point.<br><br>Hardware notes: In hardware this block costs nothing.<br><br>Example:  Suppose the input is 6 bits wide, signed, with 2 fractional bits, and the output is forced to unsigned with 0 fractional bits.  Then an input of -2.0 (1110.00 in binary 2's complement) becomes an output of 56 (111000 in binary)."
  reinterpret2 : xbsIndex_r4/Reinterpret  force_arith_type=on  arith_type=Unsigned  force_bin_pt=on  bin_pt=0  block_type=reinterpret
      settings: infoedit="Changes signal type without altering the binary representation.   You can changed the signal between signed and unsigned, and relocate the binary point.<br><br>Hardware notes: In hardware this block costs nothing.<br><br>Example:  Suppose the input is 6 bits wide, signed, with 2 fractional bits, and the output is forced to unsigned with 0 fractional bits.  Then an input of -2.0 (1110.00 in binary 2's complement) becomes an output of 56 (111000 in binary)."
  bus_out : Outport
  wires:
  concatenate/1 -> bus_out/1
  in1/1 -> reinterpret1/1
  reinterpret1/1 -> concatenate/1
  in2/1 -> reinterpret2/1
  reinterpret2/1 -> concatenate/2

== system snap_sys_clk_feng/packetizer0/header/munge_in/split ==
  bus_in : Inport
  reinterpret1 : xbsIndex_r4/Reinterpret  force_arith_type=on  arith_type=Unsigned  force_bin_pt=on  bin_pt=0  block_type=reinterpret
  reinterpret2 : xbsIndex_r4/Reinterpret  force_arith_type=on  arith_type=Unsigned  force_bin_pt=on  bin_pt=0  block_type=reinterpret
  slice1 : xbsIndex_r4/Slice  nbits=32  boolean_output=off  mode=Upper Bit Location + Width  bit1=-32  base1=MSB of Input  bit0=0  base0=LSB of Input  dbl_ovrd=off  block_type=slice
  slice2 : xbsIndex_r4/Slice  nbits=32  boolean_output=off  mode=Upper Bit Location + Width  bit1=0  base1=MSB of Input  bit0=0  base0=LSB of Input  dbl_ovrd=off  block_type=slice
  msb_out2 : Outport
  lsb_out1 : Outport  Port=2
  wires:
  bus_in/1 -> slice2/1, slice1/1
  slice2/1 -> reinterpret2/1
  reinterpret2/1 -> msb_out2/1
  slice1/1 -> reinterpret1/1
  reinterpret1/1 -> lsb_out1/1

== system snap_sys_clk_feng/packetizer0/header/munge_out/join ==
  in1 : Inport
  in2 : Inport  Port=2
  concatenate : xbsIndex_r4/Concat  num_inputs=2  dbl_ovrd=off  block_type=concat
  reinterpret1 : xbsIndex_r4/Reinterpret  force_arith_type=on  arith_type=Unsigned  force_bin_pt=on  bin_pt=0  block_type=reinterpret
      settings: infoedit="Changes signal type without altering the binary representation.   You can changed the signal between signed and unsigned, and relocate the binary point.<br><br>Hardware notes: In hardware this block costs nothing.<br><br>Example:  Suppose the input is 6 bits wide, signed, with 2 fractional bits, and the output is forced to unsigned with 0 fractional bits.  Then an input of -2.0 (1110.00 in binary 2's complement) becomes an output of 56 (111000 in binary)."
  reinterpret2 : xbsIndex_r4/Reinterpret  force_arith_type=on  arith_type=Unsigned  force_bin_pt=on  bin_pt=0  block_type=reinterpret
      settings: infoedit="Changes signal type without altering the binary representation.   You can changed the signal between signed and unsigned, and relocate the binary point.<br><br>Hardware notes: In hardware this block costs nothing.<br><br>Example:  Suppose the input is 6 bits wide, signed, with 2 fractional bits, and the output is forced to unsigned with 0 fractional bits.  Then an input of -2.0 (1110.00 in binary 2's complement) becomes an output of 56 (111000 in binary)."
  bus_out : Outport
  wires:
  concatenate/1 -> bus_out/1
  in1/1 -> reinterpret1/1
  reinterpret1/1 -> concatenate/1
  in2/1 -> reinterpret2/1
  reinterpret2/1 -> concatenate/2

== system snap_sys_clk_feng/packetizer0/header/munge_out/split ==
  bus_in : Inport
  reinterpret1 : xbsIndex_r4/Reinterpret  force_arith_type=on  arith_type=Unsigned  force_bin_pt=on  bin_pt=0  block_type=reinterpret
  reinterpret2 : xbsIndex_r4/Reinterpret  force_arith_type=on  arith_type=Unsigned  force_bin_pt=on  bin_pt=0  block_type=reinterpret
  slice1 : xbsIndex_r4/Slice  nbits=32  boolean_output=off  mode=Upper Bit Location + Width  bit1=-32  base1=MSB of Input  bit0=0  base0=LSB of Input  dbl_ovrd=off  block_type=slice
  slice2 : xbsIndex_r4/Slice  nbits=32  boolean_output=off  mode=Upper Bit Location + Width  bit1=0  base1=MSB of Input  bit0=0  base0=LSB of Input  dbl_ovrd=off  block_type=slice
  msb_out2 : Outport
  lsb_out1 : Outport  Port=2
  wires:
  bus_in/1 -> slice2/1, slice1/1
  slice2/1 -> reinterpret2/1
  reinterpret2/1 -> msb_out2/1
  slice1/1 -> reinterpret1/1
  reinterpret1/1 -> lsb_out1/1

== system snap_sys_clk_feng/packetizer1/header/munge_in/join ==
  in1 : Inport
  in2 : Inport  Port=2
  concatenate : xbsIndex_r4/Concat  num_inputs=2  dbl_ovrd=off  block_type=concat
  reinterpret1 : xbsIndex_r4/Reinterpret  force_arith_type=on  arith_type=Unsigned  force_bin_pt=on  bin_pt=0  block_type=reinterpret
      settings: infoedit="Changes signal type without altering the binary representation.   You can changed the signal between signed and unsigned, and relocate the binary point.<br><br>Hardware notes: In hardware this block costs nothing.<br><br>Example:  Suppose the input is 6 bits wide, signed, with 2 fractional bits, and the output is forced to unsigned with 0 fractional bits.  Then an input of -2.0 (1110.00 in binary 2's complement) becomes an output of 56 (111000 in binary)."
  reinterpret2 : xbsIndex_r4/Reinterpret  force_arith_type=on  arith_type=Unsigned  force_bin_pt=on  bin_pt=0  block_type=reinterpret
      settings: infoedit="Changes signal type without altering the binary representation.   You can changed the signal between signed and unsigned, and relocate the binary point.<br><br>Hardware notes: In hardware this block costs nothing.<br><br>Example:  Suppose the input is 6 bits wide, signed, with 2 fractional bits, and the output is forced to unsigned with 0 fractional bits.  Then an input of -2.0 (1110.00 in binary 2's complement) becomes an output of 56 (111000 in binary)."
  bus_out : Outport
  wires:
  reinterpret2/1 -> concatenate/2
  in2/1 -> reinterpret2/1
  reinterpret1/1 -> concatenate/1
  in1/1 -> reinterpret1/1
  concatenate/1 -> bus_out/1

== system snap_sys_clk_feng/packetizer1/header/munge_in/split ==
  bus_in : Inport
  reinterpret1 : xbsIndex_r4/Reinterpret  force_arith_type=on  arith_type=Unsigned  force_bin_pt=on  bin_pt=0  block_type=reinterpret
  reinterpret2 : xbsIndex_r4/Reinterpret  force_arith_type=on  arith_type=Unsigned  force_bin_pt=on  bin_pt=0  block_type=reinterpret
  slice1 : xbsIndex_r4/Slice  nbits=32  boolean_output=off  mode=Upper Bit Location + Width  bit1=-32  base1=MSB of Input  bit0=0  base0=LSB of Input  dbl_ovrd=off  block_type=slice
  slice2 : xbsIndex_r4/Slice  nbits=32  boolean_output=off  mode=Upper Bit Location + Width  bit1=0  base1=MSB of Input  bit0=0  base0=LSB of Input  dbl_ovrd=off  block_type=slice
  msb_out2 : Outport
  lsb_out1 : Outport  Port=2
  wires:
  reinterpret1/1 -> lsb_out1/1
  slice1/1 -> reinterpret1/1
  reinterpret2/1 -> msb_out2/1
  slice2/1 -> reinterpret2/1
  bus_in/1 -> slice1/1, slice2/1

== system snap_sys_clk_feng/packetizer1/header/munge_out/join ==
  in1 : Inport
  in2 : Inport  Port=2
  concatenate : xbsIndex_r4/Concat  num_inputs=2  dbl_ovrd=off  block_type=concat
  reinterpret1 : xbsIndex_r4/Reinterpret  force_arith_type=on  arith_type=Unsigned  force_bin_pt=on  bin_pt=0  block_type=reinterpret
      settings: infoedit="Changes signal type without altering the binary representation.   You can changed the signal between signed and unsigned, and relocate the binary point.<br><br>Hardware notes: In hardware this block costs nothing.<br><br>Example:  Suppose the input is 6 bits wide, signed, with 2 fractional bits, and the output is forced to unsigned with 0 fractional bits.  Then an input of -2.0 (1110.00 in binary 2's complement) becomes an output of 56 (111000 in binary)."
  reinterpret2 : xbsIndex_r4/Reinterpret  force_arith_type=on  arith_type=Unsigned  force_bin_pt=on  bin_pt=0  block_type=reinterpret
      settings: infoedit="Changes signal type without altering the binary representation.   You can changed the signal between signed and unsigned, and relocate the binary point.<br><br>Hardware notes: In hardware this block costs nothing.<br><br>Example:  Suppose the input is 6 bits wide, signed, with 2 fractional bits, and the output is forced to unsigned with 0 fractional bits.  Then an input of -2.0 (1110.00 in binary 2's complement) becomes an output of 56 (111000 in binary)."
  bus_out : Outport
  wires:
  reinterpret2/1 -> concatenate/2
  in2/1 -> reinterpret2/1
  reinterpret1/1 -> concatenate/1
  in1/1 -> reinterpret1/1
  concatenate/1 -> bus_out/1

== system snap_sys_clk_feng/packetizer1/header/munge_out/split ==
  bus_in : Inport
  reinterpret1 : xbsIndex_r4/Reinterpret  force_arith_type=on  arith_type=Unsigned  force_bin_pt=on  bin_pt=0  block_type=reinterpret
  reinterpret2 : xbsIndex_r4/Reinterpret  force_arith_type=on  arith_type=Unsigned  force_bin_pt=on  bin_pt=0  block_type=reinterpret
  slice1 : xbsIndex_r4/Slice  nbits=32  boolean_output=off  mode=Upper Bit Location + Width  bit1=-32  base1=MSB of Input  bit0=0  base0=LSB of Input  dbl_ovrd=off  block_type=slice
  slice2 : xbsIndex_r4/Slice  nbits=32  boolean_output=off  mode=Upper Bit Location + Width  bit1=0  base1=MSB of Input  bit0=0  base0=LSB of Input  dbl_ovrd=off  block_type=slice
  msb_out2 : Outport
  lsb_out1 : Outport  Port=2
  wires:
  reinterpret1/1 -> lsb_out1/1
  slice1/1 -> reinterpret1/1
  reinterpret2/1 -> msb_out2/1
  slice2/1 -> reinterpret2/1
  bus_in/1 -> slice1/1, slice2/1
